simulink model "apf_waypoint_offline"  (R2022b)
settings: Solver=VariableStepAuto  StartTime=0.0  StopTime=40  RelTol=1e-3
values from neighbouring files (symbols this model uses):
  e_3 = [0 0 1]'    [apf_waypoint_offline_script.m]
  g = 9.81    [apf_waypoint_offline_script.m]
  Ib = diag([0.0347563 0.0458929 0.0977])    [apf_waypoint_offline_script.m]
  Kp = diag([70 70 70])    [apf_waypoint_offline_script.m]
  Kr = diag([10 10 1.5])    [apf_waypoint_offline_script.m]
  Kv = diag([6 6 6])    [apf_waypoint_offline_script.m]
  Kw = diag([4 5.2 1.8])    [apf_waypoint_offline_script.m]
  lin_vel_0 = [0 0 0]    [waypoints_generator.m]
  mass = 1.52    [apf_waypoint_offline_script.m]
  pos_0 = q_0'    [waypoints_generator.m]
  Ts = 0.001    [apf_waypoint_offline_script.m]
  uT_0 = 14.92    [apf_waypoint_offline_script.m]
  w_bb_0 = [0 0 0]    [waypoints_generator.m]
libraries: uavsimlib x3, robotcorelib x1
settings Model: Creator=fabioruggiero  LastModifiedBy=gaetano
settings OptimizationCC: ReuseModelBlockBuffer=on
settings ModelReferenceCC: EnableRefExpFcnMdlSchedulingChecks=on

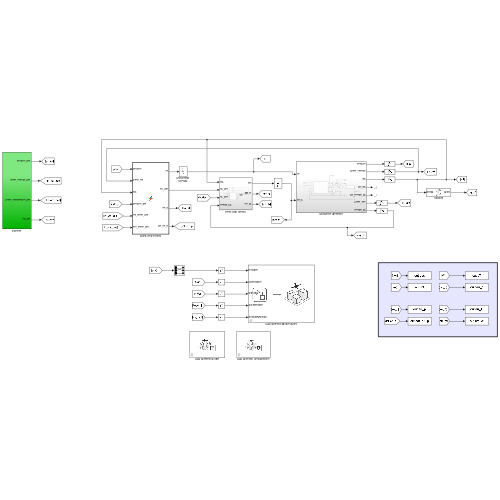
[thumbnail: Simulink's stored preview of the top-level diagram]
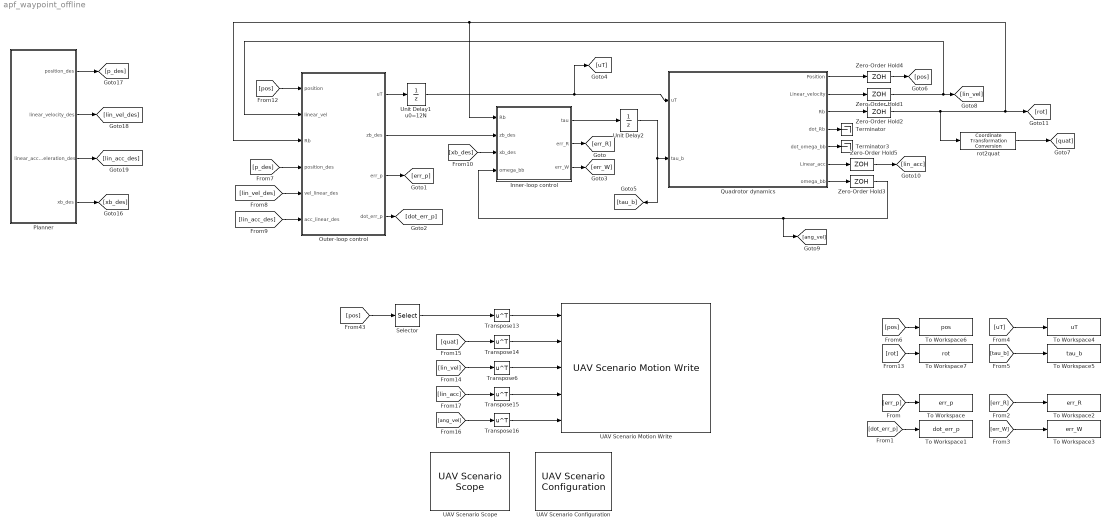
== system apf_waypoint_offline ==
  Inner-loop control : Subsystem
  Outer-loop control : MATLAB Function  TreatAsAtomicUnit=on
  Planner : Subsystem
  Quadrotor dynamics : Subsystem
  Selector : Selector  InputPortWidth=3  IndexOptions=Index vector (dialog)  Indices=[2 1 3]  OutputSizes=1
  Terminator : Terminator
  Terminator3 : Terminator
  To Workspace : ToWorkspace  VariableName=err_p  SaveFormat=Timeseries  SampleTime=-1
  To Workspace1 : ToWorkspace  VariableName=dot_err_p  SaveFormat=Timeseries  SampleTime=-1
  To Workspace2 : ToWorkspace  VariableName=err_R  SaveFormat=Timeseries  SampleTime=-1
  To Workspace3 : ToWorkspace  VariableName=err_W  SaveFormat=Timeseries  SampleTime=-1
  To Workspace4 : ToWorkspace  VariableName=uT  SaveFormat=Timeseries  SampleTime=-1
  To Workspace5 : ToWorkspace  VariableName=tau_b  SaveFormat=Timeseries  SampleTime=-1
  To Workspace6 : ToWorkspace  VariableName=pos  SaveFormat=Timeseries  SampleTime=-1
  To Workspace7 : ToWorkspace  VariableName=rot  SaveFormat=Timeseries  SampleTime=-1
  Transpose{6,13..16} (5 alike) : Math  Operator=transpose
  UAV Scenario Configuration : uavsimlib/UAV Scenario Configuration  Priority=-1  UAVScenarioObject=scene  SampleTime=0.01  UpdateParam=false  SensorMotionBusName='SensorMotionBus'  PlatformMotionBusName='PlatformMotionBus'  ScenarioMotionBusName='ScenarioMotionBus'  ScenarioMotionSignalName='ScenarioMotions'
  UAV Scenario Motion Write : uavsimlib/UAV Scenario Motion Write  Priority=0  PlatName='platformUAV'  ReferenceFrame=NED
  UAV Scenario Scope : uavsimlib/UAV Scenario Scope  Priority=1  SensorNameTable={}  SampleTime=0.1
  Unit Delay1 u0=12N : UnitDelay  InitialCondition=uT_0  SampleTime=Ts
  Unit Delay2 : UnitDelay  InitialCondition=[0 0 0]  SampleTime=Ts
  Zero-Order Hold{1..5} (5 alike) : ZeroOrderHold  SampleTime=Ts
  rot2quat : robotcorelib/Coordinate Transformation Conversion  InputRepresentation=Rotation Matrix  InputEulerSequence=ZYX  ShowTrVecInputPort=on  OutputRepresentation=Quaternion  OutputEulerSequence=ZYX  ShowTrVecOutputPort=on  SimulateUsing=Interpreted execution
  wires:
  Outer-loop control/1(uT) -> Unit Delay1 u0=12N/1
  Unit Delay1 u0=12N/1 -> Quadrotor dynamics/1(uT), [uT]
  Quadrotor dynamics/1(Position) -> Zero-Order Hold4/1
  Quadrotor dynamics/2(Linear_velocity) -> Zero-Order Hold1/1
  Quadrotor dynamics/3(Rb) -> Zero-Order Hold2/1
  Quadrotor dynamics/7(omega_bb) -> Zero-Order Hold3/1
  Zero-Order Hold1/1 -> Outer-loop control/2(linear_vel), [lin_vel]
  Zero-Order Hold2/1 -> rot2quat/1, Inner-loop control/1(Rb), Outer-loop control/3(Rb), [rot]
  Unit Delay2/1 -> [tau_b], Quadrotor dynamics/2(tau_b)
  Quadrotor dynamics/4(dot_Rb) -> Terminator/1
  Outer-loop control/3(err_p) -> [err_p]
  Outer-loop control/4(dot_err_p) -> [dot_err_p]
  Quadrotor dynamics/5(dot_omega_bb) -> Terminator3/1
  Outer-loop control/2(zb_des) -> Inner-loop control/2(zb_des)
  Zero-Order Hold3/1 -> Inner-loop control/4(omega_bb), [ang_vel]
  Inner-loop control/1(tau) -> Unit Delay2/1
  Inner-loop control/2(err_R) -> [err_R]
  Inner-loop control/3(err_W) -> [err_W]
  [err_p] -> To Workspace/1
  [dot_err_p] -> To Workspace1/1
  [err_R] -> To Workspace2/1
  [err_W] -> To Workspace3/1
  [uT] -> To Workspace4/1
  [tau_b] -> To Workspace5/1
  [pos] -> To Workspace6/1
  [p_des] -> Outer-loop control/4(position_des)
  [lin_vel_des] -> Outer-loop control/5(vel_linear_des)
  [lin_acc_des] -> Outer-loop control/6(acc_linear_des)
  [xb_des] -> Inner-loop control/3(xb_des)
  Zero-Order Hold4/1 -> [pos]
  [pos] -> Outer-loop control/1(position)
  [rot] -> To Workspace7/1
  Planner/1(position_des) -> [p_des]
  Planner/3(linear_acceleration_des) -> [lin_acc_des]
  Planner/2(linear_velocity_des) -> [lin_vel_des]
  Planner/4(xb_des) -> [xb_des]
  Transpose15/1 -> UAV Scenario Motion Write/4
  [quat] -> Transpose14/1
  [lin_vel] -> Transpose6/1
  [pos] -> Selector/1
  [ang_vel] -> Transpose16/1
  rot2quat/1 -> [quat]
  Transpose13/1 -> UAV Scenario Motion Write/1
  Transpose14/1 -> UAV Scenario Motion Write/2
  Quadrotor dynamics/6(Linear_acc) -> Zero-Order Hold5/1
  Zero-Order Hold5/1 -> [lin_acc]
  Transpose6/1 -> UAV Scenario Motion Write/3
  [lin_acc] -> Transpose15/1
  Transpose16/1 -> UAV Scenario Motion Write/5
  Selector/1 -> Transpose13/1

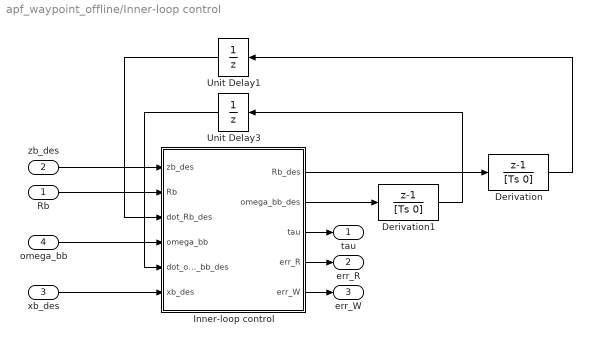
== system apf_waypoint_offline/Inner-loop control ==
  Rb : Inport
  zb_des : Inport  Port=2
  xb_des : Inport  Port=3
  omega_bb : Inport  Port=4
  Derivation : DiscreteTransferFcn  Numerator=[1 -1]  Denominator=[Ts 0]  InitialStates=[1 0 0;0 1 0;0 0 1]  SampleTime=Ts
  Derivation1 : DiscreteTransferFcn  Numerator=[1 -1]  Denominator=[Ts 0]  InitialStates=[0 0 0]  SampleTime=Ts
  Inner-loop control : MATLAB Function  TreatAsAtomicUnit=on
  Unit Delay1 : UnitDelay  InitialCondition=eye(3)  SampleTime=Ts
  Unit Delay3 : UnitDelay  InitialCondition=[0 0 0]  SampleTime=Ts
  tau : Outport
  err_R : Outport  Port=2
  err_W : Outport  Port=3
  wires:
  xb_des/1 -> Inner-loop control/6(xb_des)
  Inner-loop control/4(err_R) -> err_R/1
  Rb/1 -> Inner-loop control/2(Rb)
  Inner-loop control/3(tau) -> tau/1
  Unit Delay1/1 -> Inner-loop control/3(dot_Rb_des)
  Derivation1/1 -> Unit Delay3/1
  Inner-loop control/5(err_W) -> err_W/1
  Unit Delay3/1 -> Inner-loop control/5(dot_omega_bb_des)
  Derivation/1 -> Unit Delay1/1
  zb_des/1 -> Inner-loop control/1(zb_des)
  omega_bb/1 -> Inner-loop control/4(omega_bb)
  Inner-loop control/1(Rb_des) -> Derivation/1
  Inner-loop control/2(omega_bb_des) -> Derivation1/1

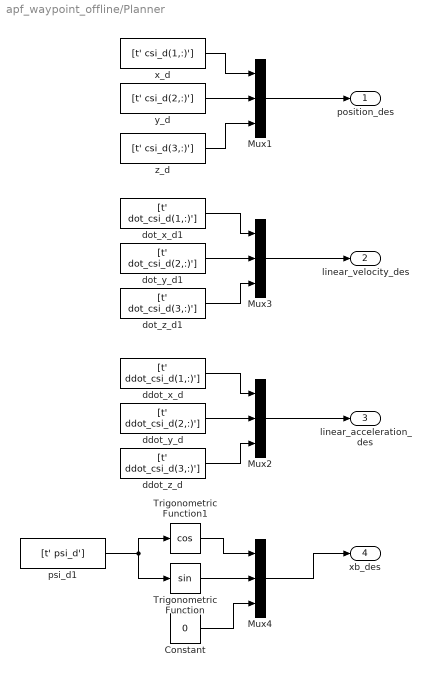
== system apf_waypoint_offline/Planner ==
  Constant : Constant  Value=0
  Mux{1..4} (4 alike) : Mux  Inputs=3
  Trigonometric Function : Trigonometry
  Trigonometric Function1 : Trigonometry  Operator=cos
  ddot_x_d : FromWorkspace  VariableName=[t' ddot_csi_d(1,:)']  SampleTime=Ts
  ddot_y_d : FromWorkspace  VariableName=[t' ddot_csi_d(2,:)']  SampleTime=Ts
  ddot_z_d : FromWorkspace  VariableName=[t' ddot_csi_d(3,:)']  SampleTime=Ts
  dot_x_d1 : FromWorkspace  VariableName=[t' dot_csi_d(1,:)']  SampleTime=Ts
  dot_y_d1 : FromWorkspace  VariableName=[t' dot_csi_d(2,:)']  SampleTime=Ts
  dot_z_d1 : FromWorkspace  VariableName=[t' dot_csi_d(3,:)']  SampleTime=Ts
  psi_d1 : FromWorkspace  VariableName=[t' psi_d']  SampleTime=Ts
  x_d : FromWorkspace  VariableName=[t' csi_d(1,:)']  SampleTime=Ts
  y_d : FromWorkspace  VariableName=[t' csi_d(2,:)']  SampleTime=Ts
  z_d : FromWorkspace  VariableName=[t' csi_d(3,:)']  SampleTime=Ts
  position_des : Outport
  linear_velocity_des : Outport  Port=2
  linear_acceleration_des : Outport  Port=3
  xb_des : Outport  Port=4
  wires:
  y_d/1 -> Mux1/2
  z_d/1 -> Mux1/3
  x_d/1 -> Mux1/1
  ddot_y_d/1 -> Mux2/2
  ddot_z_d/1 -> Mux2/3
  ddot_x_d/1 -> Mux2/1
  Mux2/1 -> linear_acceleration_des/1
  Mux1/1 -> position_des/1
  dot_y_d1/1 -> Mux3/2
  dot_z_d1/1 -> Mux3/3
  dot_x_d1/1 -> Mux3/1
  Mux3/1 -> linear_velocity_des/1
  Mux4/1 -> xb_des/1
  Trigonometric Function/1 -> Mux4/2
  psi_d1/1 -> Trigonometric Function/1, Trigonometric Function1/1
  Trigonometric Function1/1 -> Mux4/1
  Constant/1 -> Mux4/3

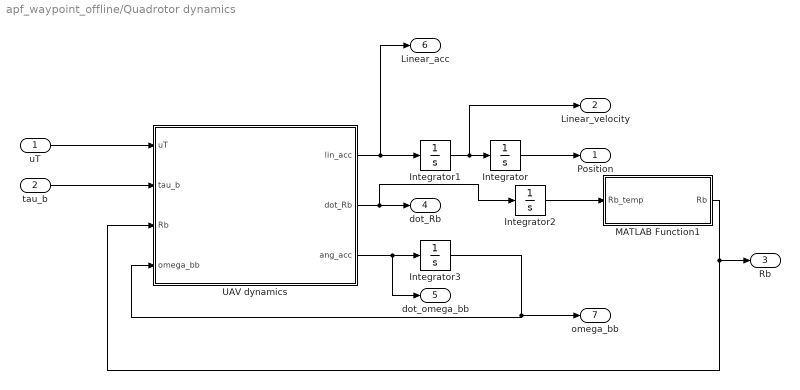
== system apf_waypoint_offline/Quadrotor dynamics ==
  uT : Inport
  tau_b : Inport  Port=2
  Integrator : Integrator  InitialCondition=pos_0
  Integrator1 : Integrator  InitialCondition=lin_vel_0
  Integrator2 : Integrator  InitialCondition=[1 0 0; 0 1 0;0 0 1]
  Integrator3 : Integrator  InitialCondition=w_bb_0
  MATLAB Function1 : MATLAB Function  TreatAsAtomicUnit=on
  UAV dynamics : MATLAB Function  TreatAsAtomicUnit=on
  Position : Outport
  Linear_velocity : Outport  Port=2
  Rb : Outport  Port=3
  dot_Rb : Outport  Port=4
  dot_omega_bb : Outport  Port=5
  Linear_acc : Outport  Port=6
  omega_bb : Outport  Port=7
  wires:
  tau_b/1 -> UAV dynamics/2(tau_b)
  Integrator/1 -> Position/1
  UAV dynamics/3(ang_acc) -> dot_omega_bb/1, Integrator3/1
  UAV dynamics/1(lin_acc) -> Linear_acc/1, Integrator1/1
  uT/1 -> UAV dynamics/1(uT)
  Integrator1/1 -> Linear_velocity/1, Integrator/1
  Integrator3/1 -> UAV dynamics/4(omega_bb), omega_bb/1
  UAV dynamics/2(dot_Rb) -> Integrator2/1, dot_Rb/1
  MATLAB Function1/1(Rb) -> Rb/1, UAV dynamics/3(Rb)
  Integrator2/1 -> MATLAB Function1/1(Rb_temp)

== matlab function apf_waypoint_offline/Quadrotor dynamics/UAV dynamics ==
  data: uT input size=1; tau_b input size=3; lin_acc output size=3; Rb input size=[3,3]; omega_bb input size=3; dot_Rb output size=[3,3]; ang_acc output size=3; mass parameter size=1; Ib parameter size=[3,3]
function [lin_acc, dot_Rb, ang_acc] = fcn(uT,tau_b,Rb,omega_bb,mass, Ib)

lin_acc = 9.81*[0 0 1]'-(uT/mass)*Rb*[0 0 1]';
dot_Rb = Rb*skew(omega_bb);
ang_acc = inv(Ib)*(-skew(omega_bb)*Ib*omega_bb + tau_b);

end

function S = skew(v)
if(numel(v)~= 1)
S= [0 -v(3) v(2); 
    v(3) 0 -v(1);
    -v(2) v(1) 0];
else
S= zeros(3);
end
end

== matlab function apf_waypoint_offline/Outer-loop control ==
  data: position input size=3; uT output size=1; linear_vel input size=3; Rb input size=[3,3]; zb_des output size=3; mass parameter size=1; position_des input size=3; vel_linear_des input size=3; acc_linear_des input size=3; err_p output size=3; dot_err_p output size=3; Kp parameter; Kv parameter; g parameter; e_3 parameter
function [uT, zb_des, err_p, dot_err_p] = fcn(position, linear_vel, Rb, mass, ...
    position_des, vel_linear_des, acc_linear_des, Kp, Kv, g, e_3)

%% WRITE HERE THE OUTER-LOOP CONTROL
% position: linear position measure
% linear_vel: linear velocity measure
% Rb: current rotation matrix
% mass: mass of the UAV
% positon_des: desired linear position from the planner
% vel_linear_des: desired linear velocity from the planner
% acc_linear_des: desired linear acceleration from the planner
% ---
% uT: commanded total thrust
% zb_des: desired z-axis of the body frame
% err_p: position error
% dot_err_p: time derivative of the positon error

%% outer loop

err_p = position - position_des;
dot_err_p = linear_vel - vel_linear_des;

uT  = -transpose(-Kp*err_p -Kv*dot_err_p -mass*g*e_3 + mass*acc_linear_des) * Rb*e_3;

zb_des = -(-Kp*err_p -Kv*dot_err_p -mass*g*e_3 + mass*acc_linear_des)/norm(-Kp*err_p -Kv*dot_err_p -mass*g*e_3 + mass*acc_linear_des);

== matlab function apf_waypoint_offline/Inner-loop control/Inner-loop control ==
  data: Rb_des output size=[3,3]; omega_bb_des output size=3; tau output size=3; zb_des input size=3; Rb input size=[3,3]; dot_Rb_des input size=[3,3]; omega_bb input size=3; dot_omega_bb_des input size=3; xb_des input size=3; Ib parameter size=[3,3]; err_R output size=3; err_W output size=3; Kr parameter; Kw parameter
function [Rb_des,omega_bb_des,tau,err_R,err_W] = fcn(zb_des,Rb,dot_Rb_des,omega_bb,dot_omega_bb_des,xb_des,Ib, Kr, Kw)

%% WRITE HERE THE INNER-LOOP CONTROL
% zb_des: desired z-axis of the body frame
% Rb: current rotation matrix
% dot_Rb_des: time-derivative of the desired rotation matrix
% omega_bb: current angular velocity expressed in the body frame
% dot_omega_bb_des: desired angular acceleration expressed in the body
% frame
% xb_des: desired x-axis of the body frame form the planner
% Ib: inertia matrix of the UAV with respect to the body frame
% ---
% Rb_des: desired rotation matrix
% omega_bb_des: desired angular velocity expressed in the body frame (given
% below as a hint)
% tau: commanded control torque
% err_R: rotational error in SO(3)
% err_W: angular velocity error in SO(3)

yb_des = (skew(zb_des)*xb_des)/norm(skew(zb_des)*xb_des);

Rb_des = [skew(yb_des)*zb_des yb_des zb_des];
omega_bb_des = wedge(Rb_des'*dot_Rb_des);

err_R = wedge(transpose(Rb_des)*Rb - transpose(Rb)*Rb_des);
err_W = omega_bb - transpose(Rb)*Rb_des*omega_bb_des;

tau = -Kr*err_R - Kw*err_W + skew(omega_bb)*Ib*omega_bb - Ib*(skew(omega_bb)*transpose(Rb)*Rb_des*omega_bb_des - transpose(Rb)*Rb_des*dot_omega_bb_des);


end

function S = skew(v)
if(numel(v)~= 1)
S= [0 -v(3) v(2); 
    v(3) 0 -v(1);
    -v(2) v(1) 0];
else
S= zeros(3);
end
end

function v = wedge(S)
v1 = S(3,2);
v2 = S(1,3);
v3 = S(2,1);
v = [v1 v2 v3]';
end

== matlab function apf_waypoint_offline/Quadrotor dynamics/MATLAB Function1 ==
  data: Rb_temp input; Rb output
function Rb = fcn(Rb_temp)
    [U,S,V] = svd(Rb_temp);
    sigma = det(U*V');
    S_ = diag([1 1 sigma]);

    Rb = U*S_*V';
end
